simulink model "dc_leg"  (R2026a)
settings: Solver=ode15s  StopTime=p.T  MaxStep=0.001  RelTol=1e-6  AbsTol=1e-8
model workspace (MAT data in the model file):
  p.M = 10
  p.m = 0.5
  p.L = 0.16
  p.width = 0.01
  p.lc = 0.08
  p.J = 0.00427083333333
  p.q0 = 1.0471975512
  p.g = 9.81
  p.torque = 8
  p.b = 11
  p.Kt = 1
  p.Ke = 1
  p.R = 1
  p.Le = 0.01
  p.Vmax = 24
  p.Kp = 5
  p.Ki = 100
  p.kGround = 100000
  p.dGround = 500
  p.transition = 0.0001
  p.T = 3
  p.Ts = 0.001
  p.z0 = 0.137583064606
  p.I0 = 7.6518
values from neighbouring files (symbols this model uses):
  p = leg_parameters    [build_leg_model.m]    (also in run_simulation.m = getVariable(get_param('dc_leg','ModelWorkspace'),'p'))
undefined symbols (not defined in the file or in its folder): X, Y, Z
libraries: sm_lib x12, nesl_utility x7
settings Model: Creator=benso  LastModifiedBy=benso

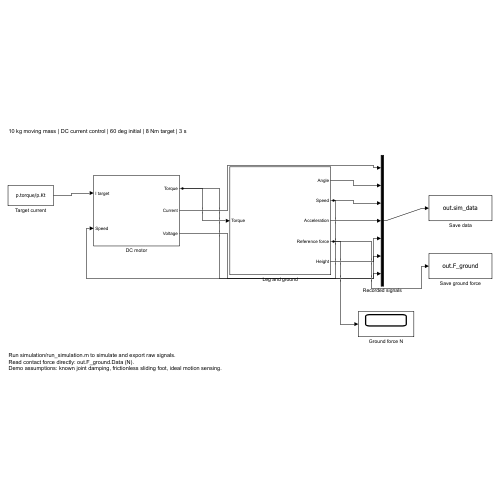
[thumbnail: Simulink's stored preview of the top-level diagram]
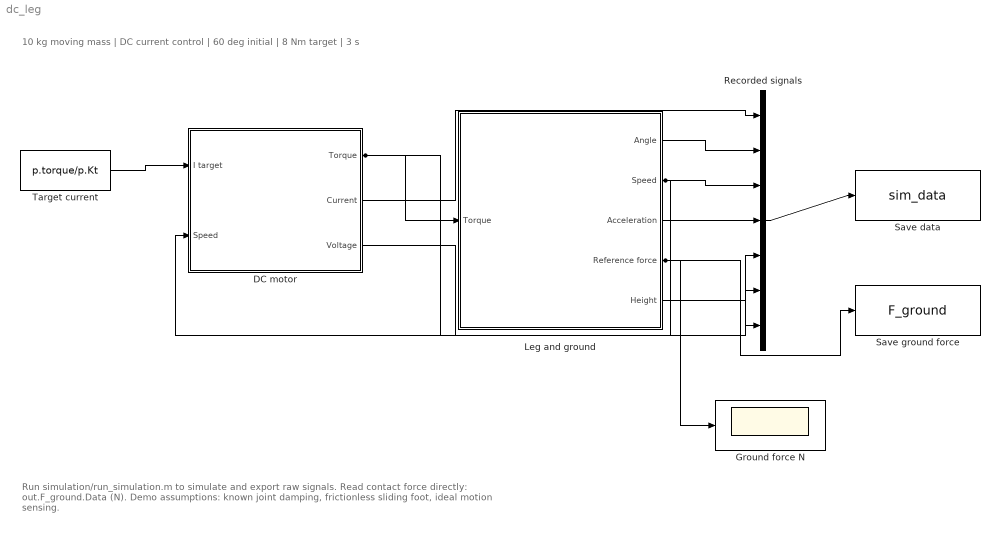
== system dc_leg ==
  note: 10 kg moving mass | DC current control | 60 deg initial | 8 Nm target | 3 s
  note: Run simulation/run_simulation.m to simulate and export raw signals.
      | Read contact force directly: out.F_ground.Data (N).
      | Demo assumptions: known joint damping, frictionless sliding foot, ideal motion sensing.
  DC motor : Subsystem
  Ground force N : Scope
  Leg and ground : Subsystem
  Recorded signals : Mux  Inputs=7
  Save data : ToWorkspace  VariableName=sim_data  SaveFormat=Timeseries  SampleTime=p.Ts
  Save ground force : ToWorkspace  VariableName=F_ground  SaveFormat=Timeseries  SampleTime=p.Ts
  Target current : Constant  Value=p.torque/p.Kt
  wires:
  Target current/1 -> DC motor/1(I target)
  DC motor/1(Torque) -> Leg and ground/1(Torque), Recorded signals/7
  Leg and ground/2(Speed) -> DC motor/2(Speed), Recorded signals/3
  DC motor/2(Current) -> Recorded signals/1
  Leg and ground/1(Angle) -> Recorded signals/2
  Leg and ground/3(Acceleration) -> Recorded signals/4
  Leg and ground/5(Height) -> Recorded signals/5
  DC motor/3(Voltage) -> Recorded signals/6
  Recorded signals/1 -> Save data/1
  Leg and ground/4(Reference force) -> Save ground force/1, Ground force N/1

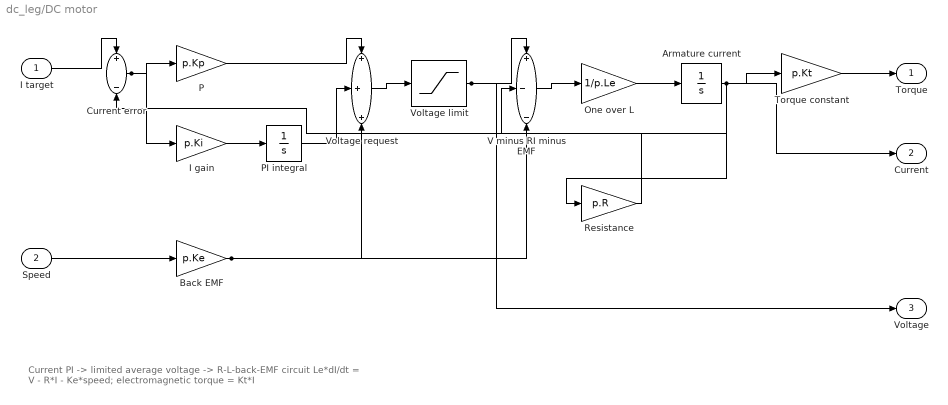
== system dc_leg/DC motor ==
  note: Current PI -> limited average voltage -> R-L-back-EMF circuit
      | Le*dI/dt = V - R*I - Ke*speed; electromagnetic torque = Kt*I
  I target : Inport
  Speed : Inport  Port=2
  Armature current : Integrator  InitialCondition=p.I0
  Back EMF : Gain  Gain=p.Ke
  Current error : Sum  Inputs=+-
  I gain : Gain  Gain=p.Ki
  One over L : Gain  Gain=1/p.Le
  P : Gain  Gain=p.Kp
  PI integral : Integrator  InitialCondition=p.R*p.I0  LimitOutput=on  UpperSaturationLimit=p.Vmax  LowerSaturationLimit=-p.Vmax
  Resistance : Gain  Gain=p.R
  Torque constant : Gain  Gain=p.Kt
  V minus RI minus EMF : Sum  Inputs=+--
  Voltage limit : Saturate  UpperLimit=p.Vmax  LowerLimit=-p.Vmax
  Voltage request : Sum  Inputs=+++
  Torque : Outport
  Current : Outport  Port=2
  Voltage : Outport  Port=3
  wires:
  I target/1 -> Current error/1
  Armature current/1 -> Current error/2, Resistance/1, Torque constant/1, Current/1
  Current error/1 -> P/1, I gain/1
  I gain/1 -> PI integral/1
  P/1 -> Voltage request/1
  PI integral/1 -> Voltage request/2
  Speed/1 -> Back EMF/1
  Back EMF/1 -> Voltage request/3, V minus RI minus EMF/3
  Voltage request/1 -> Voltage limit/1
  Voltage limit/1 -> V minus RI minus EMF/1, Voltage/1
  Resistance/1 -> V minus RI minus EMF/2
  V minus RI minus EMF/1 -> One over L/1
  One over L/1 -> Armature current/1
  Torque constant/1 -> Torque/1

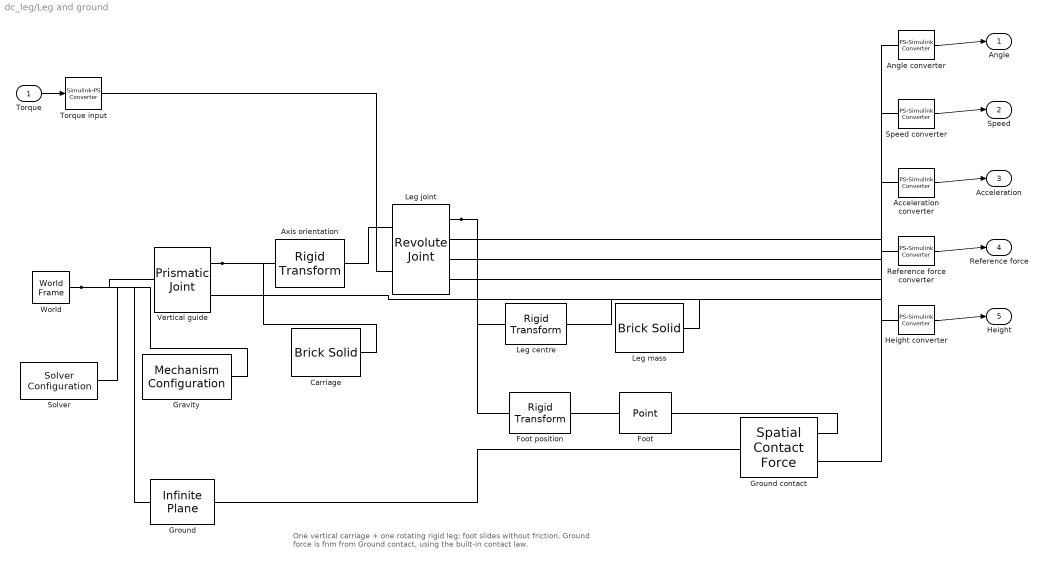
== system dc_leg/Leg and ground ==
  note: One vertical carriage + one rotating rigid leg; foot slides without friction.
      | Ground force is fnm from Ground contact, using the built-in contact law.
  Torque : Inport
  Acceleration converter : nesl_utility/PS-Simulink Converter  PhysicalDomain=network_engine_domain  SubClassName=ps_output  LeftPortType=input  RightPortType=output  PseudoPeriodic=off  Frequencies=[]  VectorFormat=inherit  Unit=rad/s^2  AffineConversion=off
  Angle converter : nesl_utility/PS-Simulink Converter  PhysicalDomain=network_engine_domain  SubClassName=ps_output  LeftPortType=input  RightPortType=output  PseudoPeriodic=off  Frequencies=[]  VectorFormat=inherit  Unit=rad  AffineConversion=off
  Axis orientation : sm_lib/Frames and Transforms/Rigid Transform  RotationMethod=StandardAxis  FollAlignAxisA=+X  BaseAlignAxisA=+Y  FollAlignAxisB=+Y  BaseAlignAxisB=+Z  RotationStandardAxis=+X  RotationAngle=-90  RotationAngleUnits=deg  RotationArbitraryAxis=[0 0 1]  RotationSequenceAxes=FollowerAxes  RotationSequence=XYX  RotationSequenceAngles=[0 0 0]  RotationSequenceAnglesUnits=deg  RotationMatrix=[1 0 0;0 1 0;0 0 1]  Quaternion=[1 0 0 0]  TranslationMethod=None  TranslationCartesianOffset=[0 0 0]  TranslationCartesianOffsetUnits=m  TranslationStandardAxis=+Z  TranslationStandardOffset=0  TranslationStandardOffsetUnits=m  TranslationROffset=0  TranslationROffsetUnits=m  TranslationThetaOffset=0  TranslationThetaOffsetUnits=deg  TranslationZOffset=0  TranslationZOffsetUnits=m
  Carriage : sm_lib/Body Elements/Brick Solid  BrickDimensions=[0.10 0.08 0.06]  BrickDimensionsUnits=m  ExportEntireGeometry=off  InertiaType=CalculateFromGeometry  BasedOnType=Mass  Density=1000  DensityUnits=kg/m^3  Mass=p.M-p.m  MassUnits=kg  CenterOfMass=[0 0 0]  CenterOfMassUnits=m  MomentsOfInertia=[1 1 1]  MomentsOfInertiaUnits=kg*m^2  ProductsOfInertia=[0 0 0]  ProductsOfInertiaUnits=kg*m^2  GraphicType=FromGeometry  MarkerShape=Sphere  MarkerSize=10  GraphicVisPropType=SimpleVisualProperties  GraphicDiffuseColor=[0.2 0.4 0.8]  GraphicOpacity=1  GraphicSpecularColor=[0.5 0.5 0.5 1.0]  GraphicAmbientColor=[0.15 0.15 0.15 1.0]  GraphicEmissiveColor=[0.0 0.0 0.0 1.0]  GraphicShininess=75  DoExposeReferenceFrame=on  SerializedFrames=<Frames/>
  Foot : sm_lib/Curves and Surfaces/Point  GraphicType=Marker  MarkerShape=Sphere  MarkerSize=4  GraphicVisPropType=SimpleVisualProperties  GraphicDiffuseColor=[0.5 0.5 0.5]  GraphicOpacity=1  GraphicSpecularColor=[0.5 0.5 0.5 1.0]  GraphicAmbientColor=[0.15 0.15 0.15 1.0]  GraphicEmissiveColor=[0.0 0.0 0.0 1.0]  GraphicShininess=75
  Foot position : sm_lib/Frames and Transforms/Rigid Transform  RotationMethod=None  FollAlignAxisA=+X  BaseAlignAxisA=+Y  FollAlignAxisB=+Y  BaseAlignAxisB=+Z  RotationStandardAxis=+Z  RotationAngle=0  RotationAngleUnits=deg  RotationArbitraryAxis=[0 0 1]  RotationSequenceAxes=FollowerAxes  RotationSequence=XYX  RotationSequenceAngles=[0 0 0]  RotationSequenceAnglesUnits=deg  RotationMatrix=[1 0 0;0 1 0;0 0 1]  Quaternion=[1 0 0 0]  TranslationMethod=Cartesian  TranslationCartesianOffset=[p.L 0 0]  TranslationCartesianOffsetUnits=m  TranslationStandardAxis=+Z  TranslationStandardOffset=0  TranslationStandardOffsetUnits=m  TranslationROffset=0  TranslationROffsetUnits=m  TranslationThetaOffset=0  TranslationThetaOffsetUnits=deg  TranslationZOffset=0  TranslationZOffsetUnits=m
  Gravity : sm_lib/Utilities/Mechanism Configuration  UniformGravity=Constant  GravityVector=[0 0 -p.g]  GravityVectorUnits=m/s^2  LinearizationDelta=0.001  JointModeTransitionNonlinearIterations=2
  Ground : sm_lib/Curves and Surfaces/Infinite Plane  GraphicType=Rectangle  GraphicPlaneWidth=0.6  GraphicPlaneWidthUnits=m  GraphicPlaneHeight=0.4  GraphicPlaneHeightUnits=m  GraphicVisPropType=SimpleVisualProperties  GraphicDiffuseColor=[0.5 0.65 0.5]  GraphicOpacity=1  GraphicSpecularColor=[0.5 0.5 0.5 1.0]  GraphicAmbientColor=[0.15 0.15 0.15 1.0]  GraphicEmissiveColor=[0.0 0.0 0.0 1.0]  GraphicShininess=75
  Ground contact : sm_lib/Forces and Torques/Spatial Contact Force  SenseSeparationDistance=off  NormalForceType=SmoothSpringDamper  NormalStiffness=p.kGround  NormalStiffnessUnits=N/m  NormalDamping=p.dGround  NormalDampingUnits=N/(m/s)  NormalTransitionRegionWidth=p.transition  NormalTransitionRegionWidthUnits=m  FrictionType=None  CoefficientOfStaticFriction=0.5  CoefficientOfDynamicFriction=0.3  FrictionalCriticalVelocity=1e-3  FrictionalCriticalVelocityUnits=m/s  SenseContactSignal=off  SensePenetrationDepth=off  SenseNormalVelocity=off  SenseTangentialVelocity=off  SensingForceTorqueDirection=BaseOnFollower  SensingForceTorqueResolutionFrame=ContactFrame  SenseNormalForce=off  SenseNormalForceMagnitude=on  SenseNormalTorque=off  SenseFrictionalForce=off  SenseFrictionalForceMagnitude=off  SenseFrictionalTorque=off  SenseTotalForce=off  SenseTotalTorque=off  SenseContactBaseRotation=off  SenseContactBaseTranslation=off  SenseContactFollowerRotation=off  SenseContactFollowerTranslation=off  ZeroCrossDetectContactStartAndEnd=off
  Height converter : nesl_utility/PS-Simulink Converter  PhysicalDomain=network_engine_domain  SubClassName=ps_output  LeftPortType=input  RightPortType=output  PseudoPeriodic=off  Frequencies=[]  VectorFormat=inherit  Unit=m  AffineConversion=off
  Leg centre : sm_lib/Frames and Transforms/Rigid Transform  RotationMethod=None  FollAlignAxisA=+X  BaseAlignAxisA=+Y  FollAlignAxisB=+Y  BaseAlignAxisB=+Z  RotationStandardAxis=+Z  RotationAngle=0  RotationAngleUnits=deg  RotationArbitraryAxis=[0 0 1]  RotationSequenceAxes=FollowerAxes  RotationSequence=XYX  RotationSequenceAngles=[0 0 0]  RotationSequenceAnglesUnits=deg  RotationMatrix=[1 0 0;0 1 0;0 0 1]  Quaternion=[1 0 0 0]  TranslationMethod=Cartesian  TranslationCartesianOffset=[p.lc 0 0]  TranslationCartesianOffsetUnits=m  TranslationStandardAxis=+Z  TranslationStandardOffset=0  TranslationStandardOffsetUnits=m  TranslationROffset=0  TranslationROffsetUnits=m  TranslationThetaOffset=0  TranslationThetaOffsetUnits=deg  TranslationZOffset=0  TranslationZOffsetUnits=m
  Leg joint : sm_lib/Joints/Revolute Joint  JointMode=Normal  CompositeWrenchDir=FollowerOnBase  CompositeWrenchFrame=BaseFrame  SenseConstraintForce=off  SenseConstraintTorque=off  SenseTotalForce=off  SenseTotalTorque=off  PositionTargetSpecify=on  PositionTargetPriority=High  PositionTargetValue=p.q0  PositionTargetValueUnits=rad  VelocityTargetSpecify=on  VelocityTargetPriority=High  VelocityTargetValue=0  VelocityTargetValueUnits=deg/s  EquilibriumPosition=0  EquilibriumPositionUnits=deg  SpringStiffness=0  SpringStiffnessUnits=N*m/deg  DampingCoefficient=p.b  DampingCoefficientUnits=N*m/(rad/s)  LowerLimitSpecify=off  LowerLimitBound=-90  LowerLimitBoundUnits=deg  LowerLimitStiffness=1e4  LowerLimitStiffnessUnits=N*m/deg  LowerLimitDamping=10  LowerLimitDampingUnits=N*m/(deg/s)  LowerLimitTransitionRegionWidth=0.1  LowerLimitTransitionRegionWidthUnits=deg  UpperLimitSpecify=off  UpperLimitBound=90  UpperLimitBoundUnits=deg  UpperLimitStiffness=1e4  UpperLimitStiffnessUnits=N*m/deg  UpperLimitDamping=10  UpperLimitDampingUnits=N*m/(deg/s)  UpperLimitTransitionRegionWidth=0.1  UpperLimitTransitionRegionWidthUnits=deg  TorqueActuationMode=InputTorque  MotionActuationMode=ComputedMotion  SensePosition=on  SenseVelocity=on  SenseAcceleration=on  SenseTorqueForce=off  SenseLowerLimitTorqueForce=off  SenseUpperLimitTorqueForce=off
  Leg mass : sm_lib/Body Elements/Brick Solid  BrickDimensions=[p.L p.width p.width]  BrickDimensionsUnits=m  ExportEntireGeometry=off  InertiaType=CalculateFromGeometry  BasedOnType=Mass  Density=1000  DensityUnits=kg/m^3  Mass=p.m  MassUnits=kg  CenterOfMass=[0 0 0]  CenterOfMassUnits=m  MomentsOfInertia=[1 1 1]  MomentsOfInertiaUnits=kg*m^2  ProductsOfInertia=[0 0 0]  ProductsOfInertiaUnits=kg*m^2  GraphicType=FromGeometry  MarkerShape=Sphere  MarkerSize=10  GraphicVisPropType=SimpleVisualProperties  GraphicDiffuseColor=[0.9 0.5 0.1]  GraphicOpacity=1  GraphicSpecularColor=[0.5 0.5 0.5 1.0]  GraphicAmbientColor=[0.15 0.15 0.15 1.0]  GraphicEmissiveColor=[0.0 0.0 0.0 1.0]  GraphicShininess=75  DoExposeReferenceFrame=on  SerializedFrames=<Frames/>
  Reference force converter : nesl_utility/PS-Simulink Converter  PhysicalDomain=network_engine_domain  SubClassName=ps_output  LeftPortType=input  RightPortType=output  PseudoPeriodic=off  Frequencies=[]  VectorFormat=inherit  Unit=N  AffineConversion=off
  Solver : nesl_utility/Solver Configuration  PhysicalDomain=network_engine_domain  SubClassName=solver  LeftPortType=input  RightPortType=generic  Tones=[]  Harmonics=[]  SimulateNoise=off  Profile=off  UseLocalSampling=off  EnableSwitchedLinearOptims=on  FrequencyDomain=off  UseCCode=off  RelTol=0.001  AbsTol=0.001  MinStep=1e-09  ToWorkspace=off  RevertToSquareIcSolve=off  NumHomotopyIterations=100  PhasorMode=off  PhasorModeNumHarmonics=1  ConsistencySolver=NEWTON_XTOL_AFTER_FTOL  CanonicalOrdering=CANONICAL  OptimizeIntermediates=OPTIMIZED  IndexReductionMethod=DerivativeReplacement  DoDC=off  ResidualTolerance=1e-09  ConsistencyTolSource=GLOBAL  ConsistencyAbsTol=0.001  ConsistencyRelTol=0.001  ConsistencyTolFactor=0.001  UseLocalSolver=off  LocalSolverChoice=NE_BACKWARD_EULER_ADVANCER  ResolveIndetEquations=on  FunctionEvalNumThread=1  LocalSolverSampleTime=0.001  DoFixedCost=off  MaxNonlinIter=3  MaxModeIter=2  ComputeImpulses=off  ImpulseIterations=2  LinearAlgebra=auto  LinearAlgebraNumThread=0  EquationFormulation=NE_TIME_EF  DelaysMemoryBudget=1024  AutomaticFiltering=on  FilteringTimeConstant=0.001  PartitionStorageMethod=AS_NEEDED  PartitionMemoryBudget=1024  PartitionMethod=ROBUST  MultibodyUseLocalSolver=off  MultibodyLocalSolverChoice=ODE1  MultibodyLocalSolverSampleTime=0.001
  Speed converter : nesl_utility/PS-Simulink Converter  PhysicalDomain=network_engine_domain  SubClassName=ps_output  LeftPortType=input  RightPortType=output  PseudoPeriodic=off  Frequencies=[]  VectorFormat=inherit  Unit=rad/s  AffineConversion=off
  Torque input : nesl_utility/Simulink-PS Converter  PhysicalDomain=network_engine_domain  SubClassName=ps_input  LeftPortType=input  RightPortType=output  PseudoPeriodic=off  Frequencies=[]  NoiseDistribution=none  NoiseParameters=[]  Unit=N*m  AffineConversion=off  FilteringAndDerivatives=provide  SimscapeFilterOrder=1  InputFilterTimeConstant=0.001  UdotUserProvided=0
  Vertical guide : sm_lib/Joints/Prismatic Joint  JointMode=Normal  CompositeWrenchDir=FollowerOnBase  CompositeWrenchFrame=BaseFrame  SenseConstraintForce=off  SenseConstraintTorque=off  SenseTotalForce=off  SenseTotalTorque=off  PositionTargetSpecify=on  PositionTargetPriority=High  PositionTargetValue=p.z0  PositionTargetValueUnits=m  VelocityTargetSpecify=on  VelocityTargetPriority=High  VelocityTargetValue=0  VelocityTargetValueUnits=m/s  EquilibriumPosition=0  EquilibriumPositionUnits=m  SpringStiffness=0  SpringStiffnessUnits=N/m  DampingCoefficient=0  DampingCoefficientUnits=N/(m/s)  LowerLimitSpecify=off  LowerLimitBound=-1  LowerLimitBoundUnits=m  LowerLimitStiffness=1e6  LowerLimitStiffnessUnits=N/m  LowerLimitDamping=1e3  LowerLimitDampingUnits=N/(m/s)  LowerLimitTransitionRegionWidth=1e-4  LowerLimitTransitionRegionWidthUnits=m  UpperLimitSpecify=off  UpperLimitBound=1  UpperLimitBoundUnits=m  UpperLimitStiffness=1e6  UpperLimitStiffnessUnits=N/m  UpperLimitDamping=1e3  UpperLimitDampingUnits=N/(m/s)  UpperLimitTransitionRegionWidth=1e-4  UpperLimitTransitionRegionWidthUnits=m  TorqueActuationMode=NoTorque  MotionActuationMode=ComputedMotion  SensePosition=on  SenseVelocity=off  SenseAcceleration=off  SenseTorqueForce=off  SenseLowerLimitTorqueForce=off  SenseUpperLimitTorqueForce=off
  World : sm_lib/Frames and Transforms/World Frame
  Angle : Outport
  Speed : Outport  Port=2
  Acceleration : Outport  Port=3
  Reference force : Outport  Port=4
  Height : Outport  Port=5
  wires:
  Torque/1 -> Torque input/1
  Angle converter/1 -> Angle/1
  Speed converter/1 -> Speed/1
  Acceleration converter/1 -> Acceleration/1
  Reference force converter/1 -> Reference force/1
  Height converter/1 -> Height/1
  connections:
  Solver/RConn1 -- World/RConn1 -- Gravity/RConn1 -- Vertical guide/LConn1 -- Ground/LConn1
  Carriage/RConn1 -- Vertical guide/RConn1 -- Axis orientation/LConn1
  Axis orientation/RConn1 -- Leg joint/LConn1
  Torque input/RConn1 -- Leg joint/LConn2
  Leg centre/LConn1 -- Leg joint/RConn1 -- Foot position/LConn1
  Leg centre/RConn1 -- Leg mass/RConn1
  Foot position/RConn1 -- Foot/LConn1
  Ground/RConn1 -- Ground contact/LConn1
  Foot/RConn1 -- Ground contact/RConn1
  Leg joint/RConn2 -- Angle converter/LConn1
  Leg joint/RConn3 -- Speed converter/LConn1
  Leg joint/RConn4 -- Acceleration converter/LConn1
  Ground contact/RConn2 -- Reference force converter/LConn1
  Vertical guide/RConn2 -- Height converter/LConn1
